simulink model "source_bin"  (R2023b)
settings: Solver=FixedStepDiscrete  StartTime=0.0  StopTime=(1e5-1)*Tb  FixedStep=Tb  RelTol=1e-3
undefined symbols (not defined in the file): graine, p1, Tb
settings Model: Creator=e2507457  LastModifiedBy=e2507457

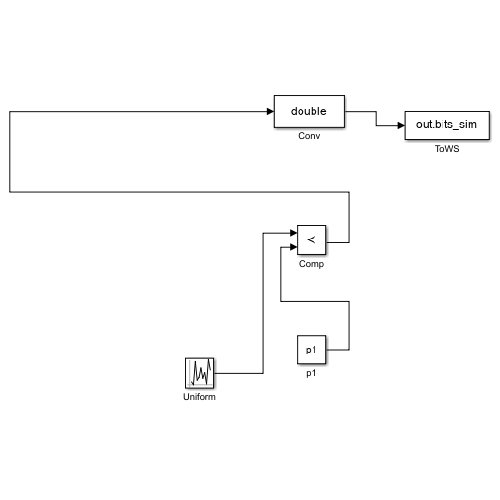
[thumbnail: Simulink's stored preview of the top-level diagram]
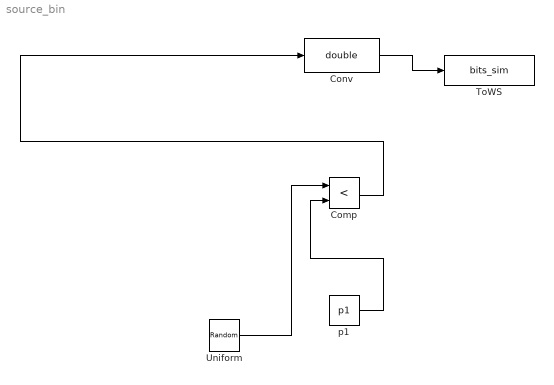
== system source_bin ==
  Comp : RelationalOperator  Operator=<  OutDataTypeStr=boolean  RndMeth=Simplest  InputSameDT=off
  Conv : DataTypeConversion  OutDataTypeStr=double  SaturateOnIntegerOverflow=off  RndMeth=Floor
  ToWS : ToWorkspace  VariableName=bits_sim  SampleTime=-1
  Uniform : UniformRandomNumber  Minimum=0  Seed=graine  SampleTime=Tb
  p1 : Constant  Value=p1  SampleTime=Tb
  wires:
  Uniform/1 -> Comp/1
  p1/1 -> Comp/2
  Comp/1 -> Conv/1
  Conv/1 -> ToWS/1
